simulink model "fm"  (R2025a)
settings: Solver=VariableStepAuto  StartTime=0.0  StopTime=0.2  MaxStep=0.0001  RelTol=1e-3
settings Model: Creator=maxaz  LastModifiedBy=LaL
settings RTWCC: GPUComputeCapability=3.5

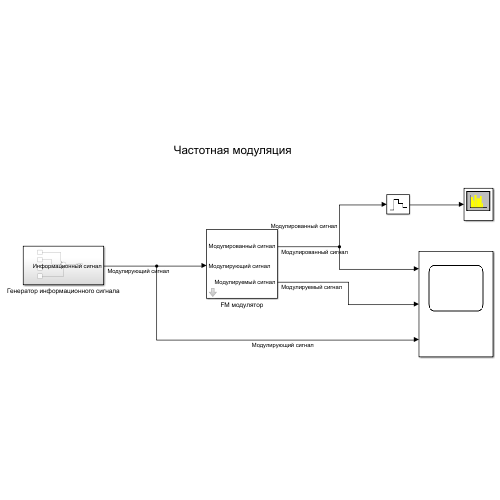
[thumbnail: Simulink's stored preview of the top-level diagram]
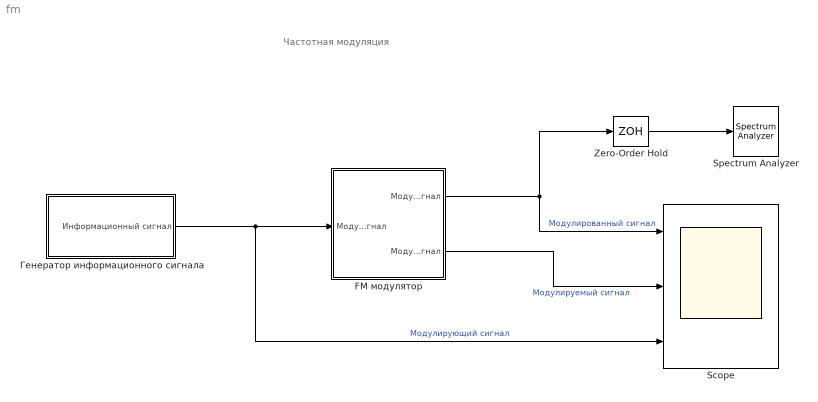
== system fm ==
  note: Частотная модуляция
  FM модулятор : Subsystem  mask{w0=300 * 2 * pi, m=100 * 2 * pi}
      mask prompts: w0 "Частота несущей"; m "Девиация фазы"
  Scope : Scope  NumInputPorts=3
      settings: ActiveDisplayYMinimum=-1.2499977582710011  ActiveDisplayYMaximum=1.2499997509190002
  Spectrum Analyzer : SpectrumAnalyzer  WindowPosition=[368.000000,230.000000,800.000000,500.000000,]  Visible=on  ScopeFrameLocation=window  Span=1000  StartFrequency=-500  StopFrequency=500  YLimits=[-68.00195555097591 46.460638080833185]  SelectedToolstripTab=spectrumAnalyzerToolstrip.measurementsTab
  Zero-Order Hold : ZeroOrderHold  SampleTime=1e-3
  Генератор информационного сигнала : Subsystem
  wires:
  Генератор информационного сигнала/1(Информационный сигнал) -> Scope/3, FM модулятор/1(Модулирующий сигнал)  "Модулирующий сигнал"
  FM модулятор/2(Модулируемый сигнал) -> Scope/2  "Модулируемый сигнал"
  Zero-Order Hold/1 -> Spectrum Analyzer/1
  FM модулятор/1(Модулированный сигнал) -> Zero-Order Hold/1, Scope/1  "Модулированный сигнал"

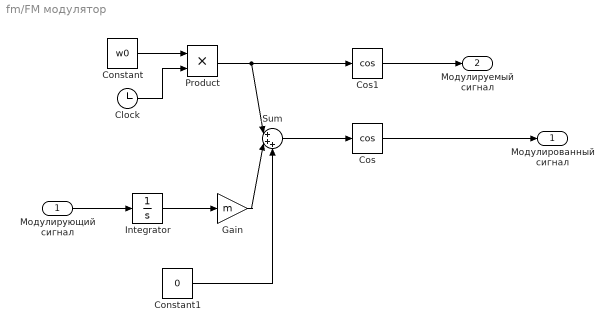
== system fm/FM модулятор ==
  Модулирующий сигнал : Inport
  Clock : Clock
  Constant : Constant  Value=w0
  Constant1 : Constant  Value=0
  Cos : Trigonometry  Operator=cos
  Cos1 : Trigonometry  Operator=cos
  Gain : Gain  Gain=m
  Integrator : Integrator
  Product : Product
  Sum : Sum  Inputs=|+++
  Модулированный сигнал : Outport
  Модулируемый сигнал : Outport  Port=2
  wires:
  Clock/1 -> Product/2
  Constant/1 -> Product/1
  Product/1 -> Sum/1, Cos1/1
  Gain/1 -> Sum/2
  Sum/1 -> Cos/1
  Cos/1 -> Модулированный сигнал/1
  Cos1/1 -> Модулируемый сигнал/1
  Модулирующий сигнал/1 -> Integrator/1
  Integrator/1 -> Gain/1
  Constant1/1 -> Sum/3

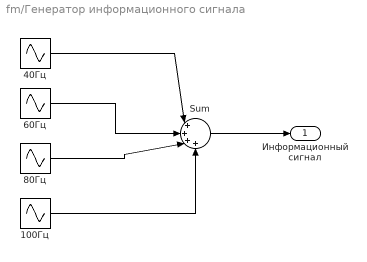
== system fm/Генератор информационного сигнала ==
  100Гц : Sin  Frequency=2*pi*100  SampleTime=0
  40Гц : Sin  Frequency=2*pi*40  SampleTime=0
  60Гц : Sin  Frequency=2*pi*60  SampleTime=0
  80Гц : Sin  Frequency=2*pi*80  SampleTime=0
  Sum : Sum  Inputs=|++++
  Информационный сигнал : Outport
  wires:
  100Гц/1 -> Sum/4
  80Гц/1 -> Sum/3
  60Гц/1 -> Sum/2
  40Гц/1 -> Sum/1
  Sum/1 -> Информационный сигнал/1
